simulink model "OpenXstim_Stage2B_Firmware"  (R2025a)
settings: Solver=FixedStepDiscrete  StartTime=0.0  StopTime=60  FixedStep=0.082500000000000004  RelTol=1e-3
settings Model: Creator=arnav  LastModifiedBy=arnav

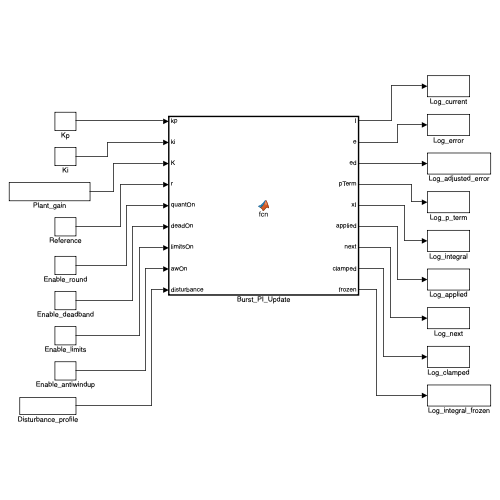
[thumbnail: Simulink's stored preview of the top-level diagram]
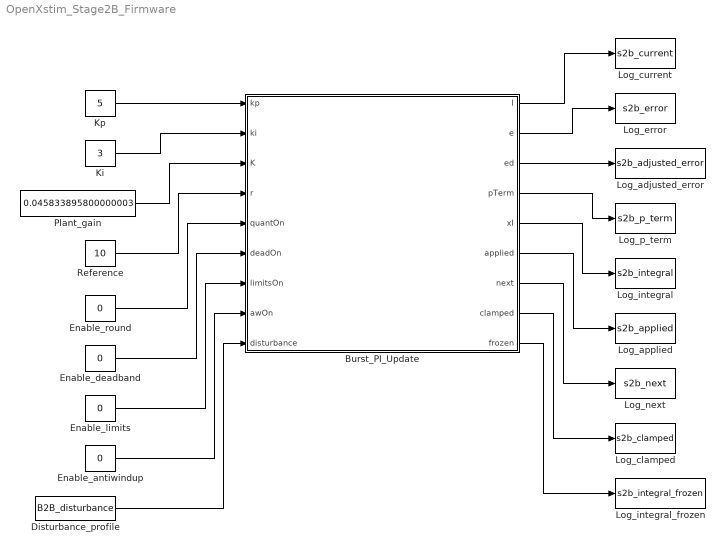
== system OpenXstim_Stage2B_Firmware ==
  Burst_PI_Update : MATLAB Function  TreatAsAtomicUnit=on
  Disturbance_profile : FromWorkspace  VariableName=B2B_disturbance  Interpolate=off  OutputAfterFinalValue=Holding final value
  Enable_antiwindup : Constant  Value=0  SampleTime=0.082500000000000004
  Enable_deadband : Constant  Value=0  SampleTime=0.082500000000000004
  Enable_limits : Constant  Value=0  SampleTime=0.082500000000000004
  Enable_round : Constant  Value=0  SampleTime=0.082500000000000004
  Ki : Constant  Value=3  SampleTime=0.082500000000000004
  Kp : Constant  Value=5  SampleTime=0.082500000000000004
  Log_adjusted_error : ToWorkspace  VariableName=s2b_adjusted_error  SaveFormat=Timeseries  SampleTime=-1
  Log_applied : ToWorkspace  VariableName=s2b_applied  SaveFormat=Timeseries  SampleTime=-1
  Log_clamped : ToWorkspace  VariableName=s2b_clamped  SaveFormat=Timeseries  SampleTime=-1
  Log_current : ToWorkspace  VariableName=s2b_current  SaveFormat=Timeseries  SampleTime=-1
  Log_error : ToWorkspace  VariableName=s2b_error  SaveFormat=Timeseries  SampleTime=-1
  Log_integral : ToWorkspace  VariableName=s2b_integral  SaveFormat=Timeseries  SampleTime=-1
  Log_integral_frozen : ToWorkspace  VariableName=s2b_integral_frozen  SaveFormat=Timeseries  SampleTime=-1
  Log_next : ToWorkspace  VariableName=s2b_next  SaveFormat=Timeseries  SampleTime=-1
  Log_p_term : ToWorkspace  VariableName=s2b_p_term  SaveFormat=Timeseries  SampleTime=-1
  Plant_gain : Constant  Value=0.045833895800000003  SampleTime=0.082500000000000004
  Reference : Constant  Value=10  SampleTime=0.082500000000000004
  wires:
  Burst_PI_Update/8(clamped) -> Log_clamped/1
  Burst_PI_Update/7(next) -> Log_next/1
  Burst_PI_Update/4(pTerm) -> Log_p_term/1
  Burst_PI_Update/3(ed) -> Log_adjusted_error/1
  Burst_PI_Update/5(xI) -> Log_integral/1
  Burst_PI_Update/1(I) -> Log_current/1
  Plant_gain/1 -> Burst_PI_Update/3(K)
  Disturbance_profile/1 -> Burst_PI_Update/9(disturbance)
  Burst_PI_Update/2(e) -> Log_error/1
  Enable_antiwindup/1 -> Burst_PI_Update/8(awOn)
  Enable_limits/1 -> Burst_PI_Update/7(limitsOn)
  Enable_deadband/1 -> Burst_PI_Update/6(deadOn)
  Burst_PI_Update/6(applied) -> Log_applied/1
  Enable_round/1 -> Burst_PI_Update/5(quantOn)
  Reference/1 -> Burst_PI_Update/4(r)
  Ki/1 -> Burst_PI_Update/2(ki)
  Burst_PI_Update/9(frozen) -> Log_integral_frozen/1
  Kp/1 -> Burst_PI_Update/1(kp)

== matlab function OpenXstim_Stage2B_Firmware/Burst_PI_Update ==
  data: kp input; I output; ki input; K input; r input; quantOn input; deadOn input; limitsOn input; awOn input; disturbance input; e output; ed output; pTerm output; xI output; applied output; next output; clamped output; frozen output
function [I,e,ed,pTerm,xI,applied,next,clamped,frozen] = fcn(kp,ki,K,r,quantOn,deadOn,limitsOn,awOn,disturbance)
%#codegen
persistent u x idx
if isempty(idx)
    idx = 0; u = 215; x = 0;
end
applied=u;
[I,e,ed,pTerm,xI,next,~,~,clamped,frozen,~] = stage2B_step( ...
    u,x,idx,kp,ki,K,9.593752,215,r,0.0825,21.5,322,25,0.03, ...
    quantOn,deadOn,limitsOn,awOn,disturbance);
u=next; x=xI; idx=idx+1;
end
